simulink model "SDA_PL_Harness_2025b"  (R2025b)
settings: Solver=FixedStepDiscrete  StartTime=0.0  StopTime=inf  FixedStep=1e-8  RelTol=1e-3
PreLoadFcn:
  | addpath('C:\Users\Cheng\Documents\MasterThesis\Model_2025b\Harness');
InitFcn:
  | setup_sda_harness_workspace_2025b;
undefined symbols (not defined in the file or in its folder): sdaHarnessAbsTol, sdaHarnessCaseLimit, sdaHarnessData, sdaHarnessRelTol
(part 2 of 2)

== stateflow chart SDA_PL_Harness_2025b/SDA_PL_Framework/SearchFSM ==
  settings: updateMethod=DISCRETE
  state IDLE
    entry: level=uint8(1); candidate=false; cycleCount=uint32(0); busy=false; resultValid=false; fault=false;
  state DONE
    entry: loadProblem=false; initStart=false; quadStart=false; vectorStart=false; memClear=false; memWrite=false; bestWrite=false; commitResult=false; busy=false; resultValid=true; fault=false;
  state FAULT
    entry: busy=false; fault=true;
  state LOAD
    entry: busy=true; loadProblem=true; memClear=true; level=uint8(1); cycleCount=uint32(0);
  state CENTER_WAIT
    during: loadProblem=false; initStart=false; quadStart=false; vectorStart=false; memClear=false; memWrite=false; bestWrite=false; commitResult=false; resultValid=false; fault=false; fsmState=uint8(6); cycleCount=cycleCount+uint32(1);
  state WRITE_RESULT
    entry: commitResult=true;
  state INIT_START
    entry: initStart=true;
  state INIT_WAIT
    during: loadProblem=false; initStart=false; quadStart=false; vectorStart=false; memClear=false; memWrite=false; bestWrite=false; commitResult=false; resultValid=false; fault=false; fsmState=uint8(3); cycleCount=cycleCount+uint32(1);
  state CENTER_START
    entry: quadStart=true;
  state SELECT_CANDIDATE
    entry: fsmState=uint8(7); candidate=quadCandidate; memWrite=true;
  state BACKTRACK
    entry: fsmState=uint8(17); if level>uint8(0); level=level-uint8(1); end; memWrite=true;
  state CHECK_LEVEL
    entry: loadProblem=false; initStart=false; quadStart=false; vectorStart=false; memClear=false; memWrite=false; bestWrite=false; commitResult=false; resultValid=false; fault=false; fsmState=uint8(4); cycleCount=cycleCount+uint32(1);
  state VECTOR_WAIT
    during: loadProblem=false; initStart=false; quadStart=false; vectorStart=false; memClear=false; memWrite=false; bestWrite=false; commitResult=false; resultValid=false; fault=false; fsmState=uint8(12); cycleCount=cycleCount+uint32(1);
  state NEXT_CANDIDATE
    entry: loadProblem=false; initStart=false; quadStart=false; vectorStart=false; memClear=false; memWrite=false; bestWrite=false; commitResult=false; resultValid=false; fault=false; fsmState=uint8(16); cycleCount=cycleCount+uint32(1);
  state DESCEND
    entry: fsmState=uint8(15); level=level+uint8(1); memWrite=true;
  state VECTOR_START
    entry: vectorStart=true;
  state VECTOR_CHECK
    entry: loadProblem=false; initStart=false; quadStart=false; vectorStart=false; memClear=false; memWrite=false; bestWrite=false; commitResult=false; resultValid=false; fault=false; fsmState=uint8(10); cycleCount=cycleCount+uint32(1);
  state UPDATE_BEST
    entry: bestWrite=true;
  state COMPARE
    entry: loadProblem=false; initStart=false; quadStart=false; vectorStart=false; memClear=false; memWrite=false; bestWrite=false; commitResult=false; resultValid=false; fault=false; fsmState=uint8(13); cycleCount=cycleCount+uint32(1);
  (default) -> IDLE
  DONE -> IDLE
  FAULT -> IDLE : [~start]
  IDLE -> LOAD : [start]
  CENTER_WAIT -> FAULT [order 2] : [quadDone && ~quadValid]
  WRITE_RESULT -> DONE
  INIT_WAIT -> FAULT [order 2] : [initDone && ~initValid]
  VECTOR_WAIT -> FAULT [order 2] : [vectorDone && ~vectorValid]
  LOAD -> INIT_START
  CENTER_WAIT -> SELECT_CANDIDATE [order 1] : [quadDone && quadValid]
  CENTER_START -> CENTER_WAIT
  INIT_START -> INIT_WAIT
  BACKTRACK -> WRITE_RESULT [order 2] : [level==uint8(0)]
  CHECK_LEVEL -> WRITE_RESULT [order 3] : [nodeLimitReached]
  INIT_WAIT -> CHECK_LEVEL [order 1] : [initDone && initValid]
  SELECT_CANDIDATE -> VECTOR_CHECK
  CHECK_LEVEL -> CENTER_START [order 1] : [~nodeLimitReached && ~candidateExhausted]
  CHECK_LEVEL -> BACKTRACK [order 2] : [~nodeLimitReached && candidateExhausted]
  BACKTRACK -> CHECK_LEVEL [order 1] : [level>uint8(0)]
  NEXT_CANDIDATE -> CHECK_LEVEL
  DESCEND -> CHECK_LEVEL
  VECTOR_WAIT -> COMPARE [order 1] : [vectorDone && vectorValid]
  VECTOR_START -> VECTOR_WAIT
  COMPARE -> NEXT_CANDIDATE [order 3] : [currentPrune || (level==uint8(15) && ~currentBetter)]
  UPDATE_BEST -> NEXT_CANDIDATE
  COMPARE -> DESCEND [order 2] : [level<uint8(15) && ~currentPrune]
  VECTOR_CHECK -> VECTOR_START [order 1] : [mod(level,uint8(3))==0]
  VECTOR_CHECK -> COMPARE [order 2] : [mod(level,uint8(3))~=0]
  COMPARE -> UPDATE_BEST [order 1] : [level==uint8(15) && currentBetter]
  data: start input boolean size=[1 1]; initDone input boolean size=[1 1]; initValid input boolean size=[1 1]; quadDone input boolean size=[1 1]; quadValid input boolean size=[1 1]; vectorDone input boolean size=[1 1]; vectorValid input boolean size=[1 1]; loadProblem output boolean size=[1 1]; initStart output boolean size=[1 1]; quadStart output boolean size=[1 1]; vectorStart output boolean size=[1 1]; memClear output boolean size=[1 1]; memWrite output boolean size=[1 1]; bestWrite output boolean size=[1 1]; commitResult output boolean size=[1 1]; busy output boolean size=[1 1]; resultValid output boolean size=[1 1]; fault output boolean size=[1 1]; level output uint8 size=[1 1]; candidate output boolean size=[1 1]; fsmState output uint8 size=[1 1]; cycleCount output uint32 size=[1 1]; quadCandidate input boolean size=[1 1]; candidateExhausted input boolean size=[1 1]; currentBetter input boolean size=[1 1]; currentPrune input boolean size=[1 1]; nodeLimitReached input boolean size=[1 1]

== matlab function SDA_PL_Harness_2025b/SDA_PL_Framework/VectorCostCalc ==
  data: problem input Bus: SdaProblemBus size=[1 1]; done output boolean size=[1 1]; start input boolean size=[1 1]; level input uint8 size=[1 1]; memory input Bus: SdaMemoryBus size=[1 1]; valid output boolean size=[1 1]; totalMetricNew output double size=[1 1]; cmvMetricNew output double size=[1 1]; cmvIncrement output double size=[1 1]; iabcNext output double size=[3 1]; deltaStep output double size=[3 1]; deltaDead output double size=[3 1]; lowerBound output double size=[3 1]; upperBound output double size=[3 1]; deadtimeMiss output boolean size=[1 1]
function [done,valid,totalMetricNew,cmvMetricNew,cmvIncrement,iabcNext,deltaStep,deltaDead,lowerBound,upperBound,deadtimeMiss] = VectorCostCalc(problem,start,level,memory)
%#codegen
persistent totalReg cmvTotalReg incrementReg iabcReg stepReg deadReg lowerReg upperReg missReg validReg startPrev doneReg
if isempty(totalReg)
    totalReg=0.0; cmvTotalReg=0.0; incrementReg=0.0;
    iabcReg=zeros(3,1); stepReg=zeros(3,1); deadReg=zeros(3,1);
    lowerReg=zeros(3,1); upperReg=zeros(3,1);
    missReg=false; validReg=false; startPrev=false; doneReg=false;
end
done=doneReg;
if start&&~startPrev
    idx=max(uint8(3),min(uint8(15),level));
    predictionStep=idivide(idx,uint8(3));
    blockEnd=double(idx); blockStart=blockEnd-2;
    sCurrent=zeros(3,1); sPrevious=zeros(3,1);
    for phase=1:3
        sCurrent(phase)=double(memory.Uwork(blockStart+phase-1));
    end
    if predictionStep==uint8(1)
        sPrevious=problem.UoptPrev(4:6);
    else
        previousStart=blockStart-3;
        for phase=1:3
            sPrevious(phase)=double(memory.Uwork(previousStart+phase-1));
        end
    end
    iabcBefore=memory.iabcPrediction(:,double(predictionStep));
    [stepReg,deadReg]=deadtime_step(sPrevious,sCurrent,iabcBefore,problem);
    [incrementReg,lowerReg,upperReg,missReg]=cmv_penalty(sPrevious,sCurrent,iabcBefore,deadReg,problem);
    totalReg=memory.metricStack(double(idx)+1)+incrementReg;
    cmvTotalReg=memory.cmvMetricStack(double(idx))+incrementReg;
    iabcReg=iabcBefore+stepReg;
    validReg=all(isfinite(iabcReg))&&isfinite(totalReg)&&isfinite(cmvTotalReg);
    doneReg=true;
end
if ~start&&~startPrev, doneReg=false; end
startPrev=start;
valid=validReg; totalMetricNew=totalReg; cmvMetricNew=cmvTotalReg;
cmvIncrement=incrementReg; iabcNext=iabcReg; deltaStep=stepReg;
deltaDead=deadReg; lowerBound=lowerReg; upperBound=upperReg;
deadtimeMiss=missReg;
end

function [deltaStep,deltaDead]=deadtime_step(sPrevious,sCurrent,iabc,problem)
sDead=sCurrent; signEps=0.1*problem.currentEpsMargin;
for phase=1:3
    if sPrevious(phase)~=sCurrent(phase)
        if iabc(phase)>=signEps
            sDead(phase)=0.0;
        elseif iabc(phase)<=-signEps
            sDead(phase)=1.0;
        elseif signEps>0.0
            sDead(phase)=0.5*(1.0-iabc(phase)/signEps);
        else
            sDead(phase)=0.5;
        end
    end
end
sEffective=problem.deadtimeRatio*sDead+(1.0-problem.deadtimeRatio)*sCurrent;
deltaDead=problem.deadtimeRatio*(problem.deltaIabcBase+problem.deltaIabcSwitch*sDead);
deltaStep=problem.deltaIabcBase+problem.deltaIabcSwitch*sEffective;
end

function [penalty,lower,upper,deadtimeMiss]=cmv_penalty(sPrevious,sCurrent,iabc,deltaDead,problem)
penalty=0.0; deadtimeMiss=false; iabcEnd=iabc+deltaDead;
lower=min(iabc,iabcEnd)-problem.currentEpsMargin;
upper=max(iabc,iabcEnd)+problem.currentEpsMargin;
uncertain=(lower<=0.0)&(upper>=0.0);
if all(sCurrent==0.0)||all(sCurrent==1.0)
    penalty=penalty+problem.lambdaZero;
end
changed=(sPrevious~=sCurrent);
if sum(changed)==2
    canZero=false(3,1); canOne=false(3,1);
    for phase=1:3
        if ~changed(phase)
            canZero(phase)=sPrevious(phase)==0.0;
            canOne(phase)=sPrevious(phase)==1.0;
        elseif uncertain(phase)
            canZero(phase)=true; canOne(phase)=true;
        elseif iabcEnd(phase)>0.0
            canZero(phase)=true;
        else
            canOne(phase)=true;
        end
    end
    deadtimeMiss=all(canZero)||all(canOne);
    if deadtimeMiss
        penalty=penalty+problem.lambdaDeadtime;
    end
end
end

== matlab function SDA_PL_Harness_2025b/AutomaticComparator ==
  data: pl input; lastPass output; ref input; enable input; absTol input; relTol input; passCount output; failCount output; comparedCount output; maxAbsError output; maxRelError output; mismatchMask output
function [lastPass,passCount,failCount,comparedCount,maxAbsError,maxRelError,mismatchMask] = fcn(pl,ref,enable,absTol,relTol)
%#codegen
persistent pCount fCount cCount maxAbs maxRel last mask
if isempty(pCount), pCount=uint32(0); fCount=uint32(0); cCount=uint32(0); maxAbs=0.0; maxRel=0.0; last=true; mask=uint32(0); end
if enable
 exactOK = isequal(pl.nodes,ref.nodes) && isequal(pl.optimal,ref.optimal) && ...
  isequal(pl.Uopt,ref.Uopt) && isequal(pl.Uapply,ref.Uapply) && ...
  isequal(pl.predictionValidNext,ref.predictionValidNext) && ...
  isequal(pl.leafNodes,ref.leafNodes) && ...
  isequal(pl.switchCountApplied,ref.switchCountApplied);
 a=[pl.Jopt;pl.iabcPredictedNext(:);pl.bestCMVCost;pl.cmvMetricRatio;pl.debug_lower(:);pl.debug_upper(:);pl.Jround;pl.Jshift];
 b=[ref.Jopt;ref.iabcPredictedNext(:);ref.bestCMVCost;ref.cmvMetricRatio;ref.debug_lower(:);ref.debug_upper(:);ref.Jround;ref.Jshift];
 e=max(abs(a-b)); scale=max(1.0,max(abs(b))); r=e/scale; floatOK=e<=absTol+relTol*scale;
 last=exactOK && floatOK; cCount=cCount+uint32(1); maxAbs=max(maxAbs,e); maxRel=max(maxRel,r);
 if last, pCount=pCount+uint32(1); else, fCount=fCount+uint32(1); end
 mask=uint32(0);
 if ~isequal(pl.nodes,ref.nodes), mask=bitor(mask,uint32(1)); end
 if ~isequal(pl.leafNodes,ref.leafNodes), mask=bitor(mask,uint32(2)); end
 if ~isequal(pl.Uopt,ref.Uopt), mask=bitor(mask,uint32(4)); end
 if ~isequal(pl.Uapply,ref.Uapply), mask=bitor(mask,uint32(8)); end
 if ~floatOK, mask=bitor(mask,uint32(16)); end
end
lastPass=last; passCount=pCount; failCount=fCount; comparedCount=cCount; maxAbsError=maxAbs; maxRelError=maxRel; mismatchMask=mask;
end
